simulink model "gnc_MissionManager"  (R2026b)
settings: Solver=VariableStepAuto
values from neighbouring files (symbols this model uses):
  Ts = prm.Ts    [gnc_missionFSM.m]    (also in gnc_mpcPlantUpdate.m)
undefined symbols (not defined in the file or in its folder): MissionType, P
libraries: simulink x1
settings Model: Creator=aomar  LastModifiedBy=aomar

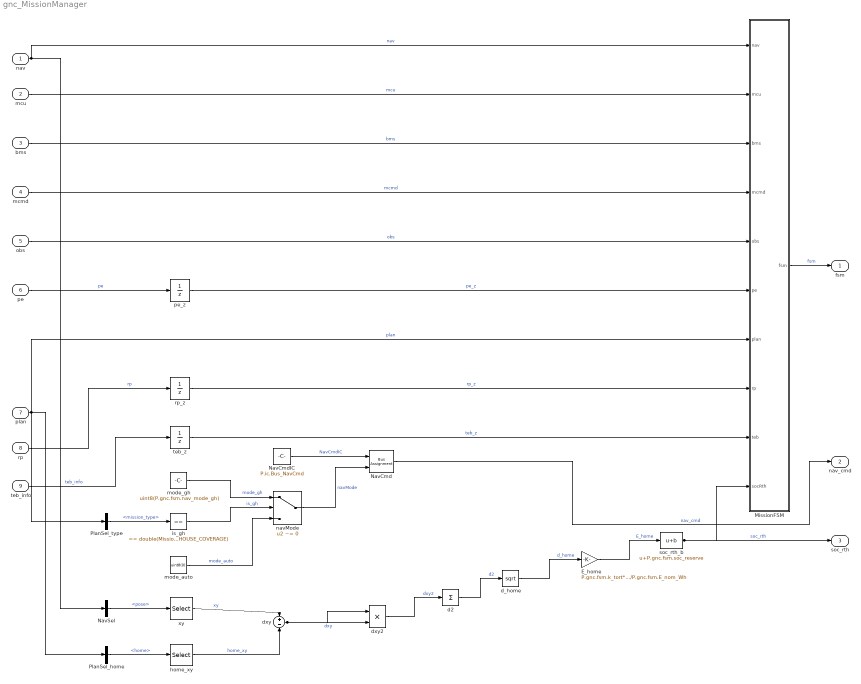
== system gnc_MissionManager ==
  nav : Inport  OutDataTypeStr=Bus: Bus_NavCond  SampleTime=Ts.gnc
  mcu : Inport  Port=2  OutDataTypeStr=Bus: Bus_McuStatus  SampleTime=Ts.gnc
  bms : Inport  Port=3  OutDataTypeStr=Bus: Bus_BmsStatus  SampleTime=Ts.gnc
  mcmd : Inport  Port=4  OutDataTypeStr=Bus: Bus_MissionCmd  SampleTime=Ts.gnc
  obs : Inport  Port=5  OutDataTypeStr=Bus: Bus_ObsFlags  SampleTime=Ts.gnc
  pe : Inport  Port=6  OutDataTypeStr=Bus: Bus_PathError  SampleTime=Ts.gnc
  plan : Inport  Port=7  OutDataTypeStr=Bus: Bus_MissionPlan
  rp : Inport  Port=8  OutDataTypeStr=Bus: Bus_ReplanResult  SampleTime=Ts.gnc
  teb_info : Inport  Port=9  OutDataTypeStr=double  PortDimensions=4  SampleTime=Ts.gnc
  E_home : Gain  Gain=P.gnc.fsm.k_tort*P.gnc.fsm.e_m*P.gnc.fsm.k_margin/P.gnc.fsm.E_nom_Wh
  MissionFSM : MATLAB Function  TreatAsAtomicUnit=on  mask{prm=P.gnc.fsm}
  NavCmd : BusAssignment  AssignedSignals=navMode
  NavCmdIC : Constant  Value=P.ic.Bus_NavCmd  OutDataTypeStr=Bus: Bus_NavCmd  SampleTime=Ts.gnc
  NavSel : BusSelector  OutputSignals=pose
  PlanSel_home : BusSelector  OutputSignals=home
  PlanSel_type : BusSelector  OutputSignals=mission_type
  d2 : Sum  Inputs=+
  d_home : Sqrt
  dxy : Sum  Inputs=+-
  dxy2 : Product  Inputs=**
  home_xy : Selector  IndexOptions=Index vector (dialog)  Indices=[1 2]  OutputSizes=1
  is_gh : simulink/Logic and Bit Operations/Compare To Constant  relop===  const=double(MissionType.GREENHOUSE_COVERAGE)  OutDataTypeStr=boolean
  mode_auto : Constant  Value=uint8(0)  OutDataTypeStr=uint8  SampleTime=Ts.gnc
  mode_gh : Constant  Value=uint8(P.gnc.fsm.nav_mode_gh)  OutDataTypeStr=uint8  SampleTime=Ts.gnc
  navMode : Switch  Criteria=u2 ~= 0  SaturateOnIntegerOverflow=off  InputSameDT=off
  pe_z : UnitDelay  InitialCondition=P.ic.Bus_PathError  SampleTime=-1
  rp_z : UnitDelay  InitialCondition=P.ic.Bus_ReplanResult  SampleTime=-1
  soc_rth_b : Bias  Bias=P.gnc.fsm.soc_reserve  SaturateOnIntegerOverflow=off
  teb_z : UnitDelay  InitialCondition=zeros(4,1)  SampleTime=-1
  xy : Selector  IndexOptions=Index vector (dialog)  Indices=[1 2]  OutputSizes=1
  fsm : Outport  OutDataTypeStr=Bus: Bus_FsmOut
  nav_cmd : Outport  Port=2  OutDataTypeStr=Bus: Bus_NavCmd
  soc_rth : Outport  Port=3  OutDataTypeStr=double
  wires:
  nav/1 -> NavSel/1, MissionFSM/1(nav)  "nav"
  mcu/1 -> MissionFSM/2(mcu)  "mcu"
  bms/1 -> MissionFSM/3(bms)  "bms"
  mcmd/1 -> MissionFSM/4(mcmd)  "mcmd"
  obs/1 -> MissionFSM/5(obs)  "obs"
  pe/1 -> pe_z/1  "pe"
  plan/1 -> PlanSel_home/1, PlanSel_type/1, MissionFSM/7(plan)  "plan"
  rp/1 -> rp_z/1  "rp"
  teb_info/1 -> teb_z/1  "teb_info"
  PlanSel_type/1 -> is_gh/1  "<mission_type>"
  NavSel/1 -> xy/1  "<pose>"
  PlanSel_home/1 -> home_xy/1  "<home>"
  mode_gh/1 -> navMode/1  "mode_gh"
  is_gh/1 -> navMode/2  "is_gh"
  mode_auto/1 -> navMode/3  "mode_auto"
  pe_z/1 -> MissionFSM/6(pe)  "pe_z"
  rp_z/1 -> MissionFSM/8(rp)  "rp_z"
  teb_z/1 -> MissionFSM/9(teb)  "teb_z"
  xy/1 -> dxy/1  "xy"
  home_xy/1 -> dxy/2  "home_xy"
  dxy/1 -> dxy2/1, dxy2/2  "dxy"
  NavCmdIC/1 -> NavCmd/1  "NavCmdIC"
  navMode/1 -> NavCmd/2  "navMode"
  dxy2/1 -> d2/1  "dxy2"
  NavCmd/1 -> nav_cmd/1  "nav_cmd"
  d2/1 -> d_home/1  "d2"
  d_home/1 -> E_home/1  "d_home"
  E_home/1 -> soc_rth_b/1  "E_home"
  soc_rth_b/1 -> MissionFSM/10(socRth), soc_rth/1  "soc_rth"
  MissionFSM/1(fsm) -> fsm/1  "fsm"

== matlab function gnc_MissionManager/MissionFSM ==
  settings: updateMethod=DISCRETE  sampleTime=Ts.gnc  description=Mission manager FSM (gnc spec 4.1, build plan T15); body subsystems/gnc/gnc_missionFSM.m.
  data: nav input Bus: Bus_NavCond; fsm output Bus: Bus_FsmOut; mcu input Bus: Bus_McuStatus; bms input Bus: Bus_BmsStatus; mcmd input Bus: Bus_MissionCmd; obs input Bus: Bus_ObsFlags; pe input Bus: Bus_PathError; plan input Bus: Bus_MissionPlan; rp input Bus: Bus_ReplanResult; teb input double; socRth input double; prm parameter
function fsm = fcn(nav, mcu, bms, mcmd, obs, pe, plan, rp, teb, socRth, prm)
%#codegen
fsm = gnc_missionFSM(nav, mcu, bms, mcmd, obs, pe, plan, rp, teb, socRth, prm);
